simulink model "block_diagram_ode1"  (R2025b)
settings: Solver=ode8  StartTime=0.0  StopTime=10.0  FixedStep=0.01  RelTol=1e-3
settings Model: Creator=MehrSystem  LastModifiedBy=MehrSystem

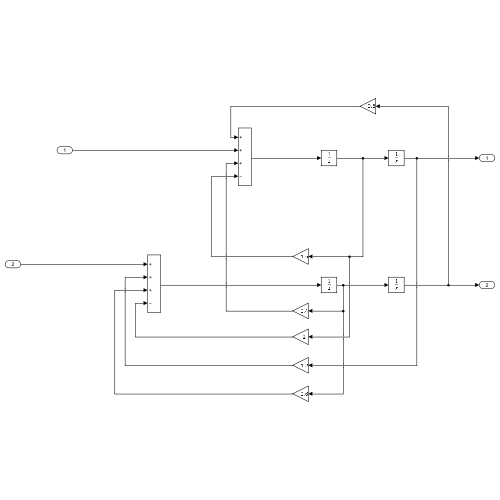
[thumbnail: Simulink's stored preview of the top-level diagram]
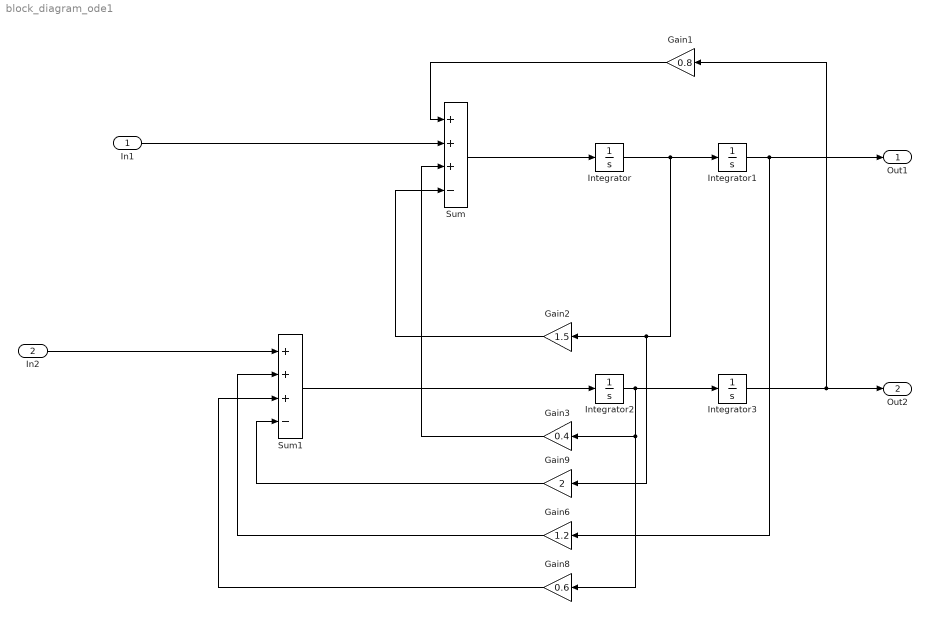
== system block_diagram_ode1 ==
  In1 : Inport
  In2 : Inport  Port=2
  Gain1 : Gain  Gain=0.8
  Gain2 : Gain  Gain=1.5
  Gain3 : Gain  Gain=0.4
  Gain6 : Gain  Gain=1.2
  Gain8 : Gain  Gain=0.6
  Gain9 : Gain  Gain=2
  Integrator{,1..3} (4 alike) : Integrator
  Sum : Sum  Inputs=+++-
  Sum1 : Sum  Inputs=+++-
  Out1 : Outport
  Out2 : Outport  Port=2
  wires:
  Integrator/1 -> Gain2/1, Gain9/1, Integrator1/1
  Integrator1/1 -> Out1/1, Gain6/1
  Integrator2/1 -> Gain3/1, Gain8/1, Integrator3/1
  Sum/1 -> Integrator/1
  Integrator3/1 -> Gain1/1, Out2/1
  Gain1/1 -> Sum/1
  Gain2/1 -> Sum/4
  Gain3/1 -> Sum/3
  In1/1 -> Sum/2
  Sum1/1 -> Integrator2/1
  In2/1 -> Sum1/1
  Gain6/1 -> Sum1/2
  Gain8/1 -> Sum1/3
  Gain9/1 -> Sum1/4
